simulink model "AXU5EV_PL_Algorithm_Library"  (R2026b)
settings: Solver=VariableStepAuto
libraries: $bdroot x2
settings Model: Creator=lww  LastModifiedBy=lww

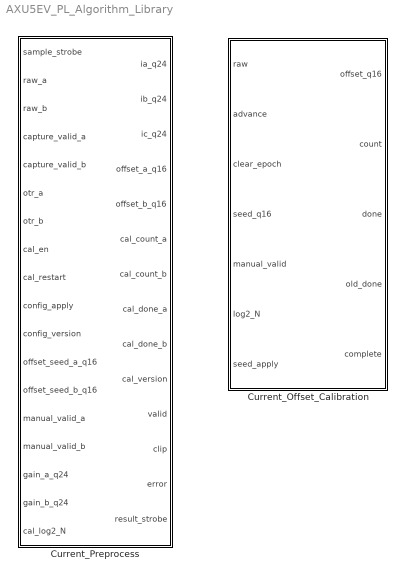
== system AXU5EV_PL_Algorithm_Library ==
  Current_Offset_Calibration : Subsystem  Description=Extracted from the AQM F28335 backup Current_Offset_Calibration (SID350). One independently qualified channel, linked twice for A/B. raw codes -> sum/count -> Q16 offset. Config seeds and log2 window are input ports. Completing sample is rejected using old_done.
  Current_Preprocess : Subsystem  Description=Task1 shared visible current graph. AN9238 Q16 offsets and signed Q24 gains remain atomic input configuration. Independent valid/OTR qualification, wide two-phase reconstruction, convergent rounding and one-clock output registers are preserved.

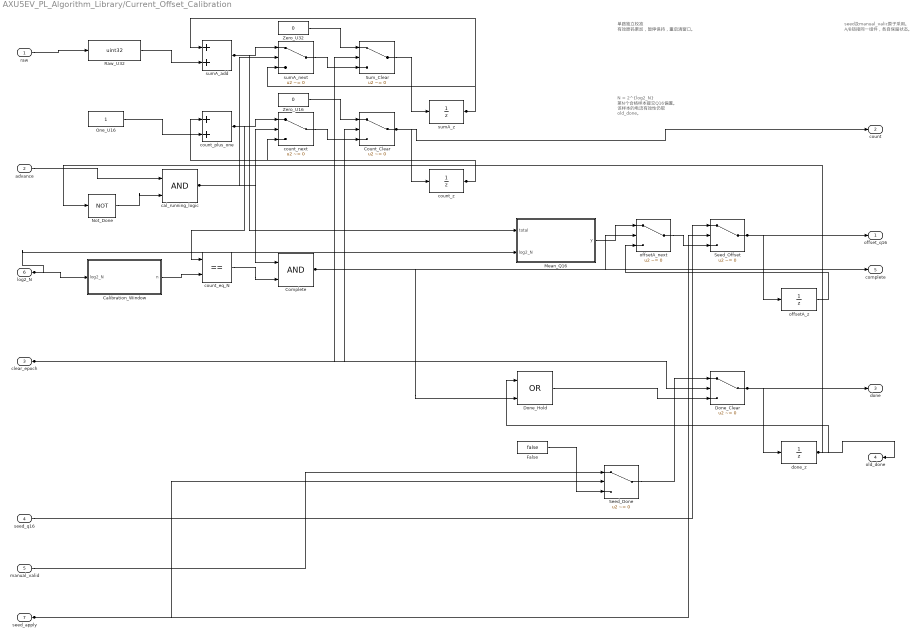
== system AXU5EV_PL_Algorithm_Library/Current_Offset_Calibration ==
  note: seed及manual_valid原子采用。
      | A/B链接同一组件，各自保留状态。
  note: N = 2^{log2_N}
      | 第N个合格样本提交Q16偏置。
      | 该样本的电流有效性仍取 old_done。
  note: 单路独立校准
      | 有效原码累加，暂停保持，重启清窗口。
  raw : Inport  OutDataTypeStr=uint16
  advance : Inport  Port=2  OutDataTypeStr=boolean
  clear_epoch : Inport  Port=3  OutDataTypeStr=boolean
  seed_q16 : Inport  Port=4  OutDataTypeStr=int32
  manual_valid : Inport  Port=5  OutDataTypeStr=boolean
  log2_N : Inport  Port=6  OutDataTypeStr=uint8
  seed_apply : Inport  Port=7  OutDataTypeStr=boolean
  Calibration_Window : MATLAB Function  TreatAsAtomicUnit=on
  Complete : Logic  IconShape=distinctive  AllPortsSameDT=off  OutDataTypeStr=boolean
  Count_Clear : Switch  Criteria=u2 ~= 0  SaturateOnIntegerOverflow=off  InputSameDT=off
  Done_Clear : Switch  Criteria=u2 ~= 0  SaturateOnIntegerOverflow=off  InputSameDT=off
  Done_Hold : Logic  Operator=OR  IconShape=distinctive  AllPortsSameDT=off  OutDataTypeStr=boolean
  False : Constant  Value=false  OutDataTypeStr=boolean
  Mean_Q16 : MATLAB Function  TreatAsAtomicUnit=on
  Not_Done : Logic  Operator=NOT  Inputs=1  IconShape=distinctive  AllPortsSameDT=off  OutDataTypeStr=boolean
  One_U16 : Constant  OutDataTypeStr=uint16
  Raw_U32 : DataTypeConversion  OutDataTypeStr=uint32  SaturateOnIntegerOverflow=off  RndMeth=Floor
  Seed_Done : Switch  Criteria=u2 ~= 0  SaturateOnIntegerOverflow=off  InputSameDT=off
  Seed_Offset : Switch  Criteria=u2 ~= 0  SaturateOnIntegerOverflow=off  InputSameDT=off
  Sum_Clear : Switch  Criteria=u2 ~= 0  SaturateOnIntegerOverflow=off  InputSameDT=off
  Zero_U16 : Constant  Value=0  OutDataTypeStr=uint16
  Zero_U32 : Constant  Value=0  OutDataTypeStr=uint32
  cal_running_logic : Logic  IconShape=distinctive  AllPortsSameDT=off  OutDataTypeStr=boolean
  count_eq_N : RelationalOperator  Operator===  OutDataTypeStr=boolean  RndMeth=Simplest  InputSameDT=off
  count_next : Switch  Criteria=u2 ~= 0  Threshold=0.5  OutDataTypeStr=uint16  SaturateOnIntegerOverflow=off  InputSameDT=off
  count_plus_one : Sum  OutDataTypeStr=uint16
  count_z : UnitDelay  SampleTime=-1
  done_z : UnitDelay  InitialCondition=false  SampleTime=-1
  offsetA_next : Switch  Criteria=u2 ~= 0  Threshold=0.5  OutDataTypeStr=int32  SaturateOnIntegerOverflow=off  InputSameDT=off
  offsetA_z : UnitDelay  SampleTime=-1
  sumA_add : Sum  OutDataTypeStr=uint32
  sumA_next : Switch  Criteria=u2 ~= 0  Threshold=0.5  OutDataTypeStr=uint32  SaturateOnIntegerOverflow=off  InputSameDT=off
  sumA_z : UnitDelay  SampleTime=-1
  offset_q16 : Outport
  count : Outport  Port=2
  done : Outport  Port=3
  old_done : Outport  Port=4
  complete : Outport  Port=5
  wires:
  Done_Clear/1 -> done_z/1, done/1
  Done_Hold/1 -> Done_Clear/3
  Seed_Done/1 -> Done_Clear/1
  False/1 -> Seed_Done/3
  manual_valid/1 -> Seed_Done/1
  Seed_Offset/1 -> offset_q16/1, offsetA_z/1
  seed_apply/1 -> Seed_Offset/2, Seed_Done/2
  seed_q16/1 -> Seed_Offset/1
  Complete/1 -> offsetA_next/2, Done_Hold/2, complete/1
  Mean_Q16/1(y) -> offsetA_next/1
  count_eq_N/1 -> Complete/2
  Calibration_Window/1(n) -> count_eq_N/2
  log2_N/1 -> Calibration_Window/1(log2_N), Mean_Q16/2(log2_N)
  Count_Clear/1 -> count_z/1, count/1
  Sum_Clear/1 -> sumA_z/1
  Zero_U16/1 -> Count_Clear/1
  clear_epoch/1 -> Count_Clear/2, Sum_Clear/2, Done_Clear/2
  Zero_U32/1 -> Sum_Clear/1
  cal_running_logic/1 -> Complete/1, sumA_next/2, count_next/2
  One_U16/1 -> count_plus_one/2
  Raw_U32/1 -> sumA_add/2
  Not_Done/1 -> cal_running_logic/2
  advance/1 -> cal_running_logic/1
  done_z/1 -> old_done/1, Not_Done/1, Done_Hold/1
  offsetA_next/1 -> Seed_Offset/3
  offsetA_z/1 -> offsetA_next/3
  sumA_next/1 -> Sum_Clear/3
  sumA_add/1 -> sumA_next/1, Mean_Q16/1(total)
  raw/1 -> Raw_U32/1
  sumA_z/1 -> sumA_add/1, sumA_next/3
  count_next/1 -> Count_Clear/3
  count_plus_one/1 -> count_next/1, count_eq_N/1
  count_z/1 -> count_plus_one/1, count_next/3

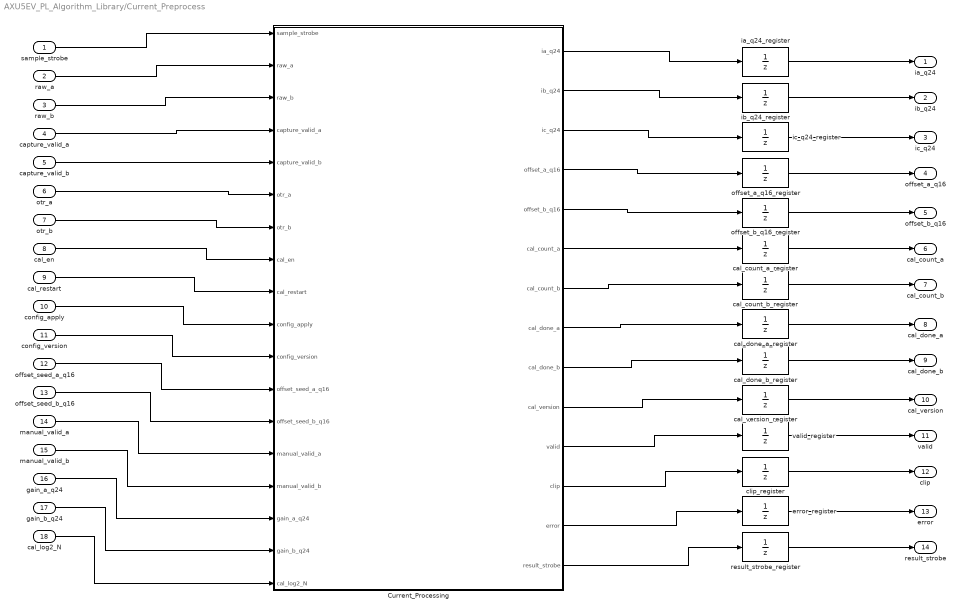
== system AXU5EV_PL_Algorithm_Library/Current_Preprocess ==
  sample_strobe : Inport  OutDataTypeStr=boolean  SampleTime=2e-8
  raw_a : Inport  Port=2  OutDataTypeStr=uint16  SampleTime=2e-8
  raw_b : Inport  Port=3  OutDataTypeStr=uint16  SampleTime=2e-8
  capture_valid_a : Inport  Port=4  OutDataTypeStr=boolean  SampleTime=2e-8
  capture_valid_b : Inport  Port=5  OutDataTypeStr=boolean  SampleTime=2e-8
  otr_a : Inport  Port=6  OutDataTypeStr=boolean  SampleTime=2e-8
  otr_b : Inport  Port=7  OutDataTypeStr=boolean  SampleTime=2e-8
  cal_en : Inport  Port=8  OutDataTypeStr=boolean  SampleTime=2e-8
  cal_restart : Inport  Port=9  OutDataTypeStr=boolean  SampleTime=2e-8
  config_apply : Inport  Port=10  OutDataTypeStr=boolean  SampleTime=2e-8
  config_version : Inport  Port=11  OutDataTypeStr=uint32  SampleTime=2e-8
  offset_seed_a_q16 : Inport  Port=12  OutDataTypeStr=int32  SampleTime=2e-8
  offset_seed_b_q16 : Inport  Port=13  OutDataTypeStr=int32  SampleTime=2e-8
  manual_valid_a : Inport  Port=14  OutDataTypeStr=boolean  SampleTime=2e-8
  manual_valid_b : Inport  Port=15  OutDataTypeStr=boolean  SampleTime=2e-8
  gain_a_q24 : Inport  Port=16  OutDataTypeStr=int32  SampleTime=2e-8
  gain_b_q24 : Inport  Port=17  OutDataTypeStr=int32  SampleTime=2e-8
  cal_log2_N : Inport  Port=18  OutDataTypeStr=uint8  SampleTime=2e-8
  Current_Processing : Subsystem
  cal_count_a_register : UnitDelay  SampleTime=-1
  cal_count_b_register : UnitDelay  SampleTime=-1
  cal_done_a_register : UnitDelay  SampleTime=-1
  cal_done_b_register : UnitDelay  SampleTime=-1
  cal_version_register : UnitDelay  SampleTime=-1
  clip_register : UnitDelay  SampleTime=-1
  error_register : UnitDelay  SampleTime=-1
  ia_q24_register : UnitDelay  SampleTime=-1
  ib_q24_register : UnitDelay  SampleTime=-1
  ic_q24_register : UnitDelay  SampleTime=-1
  offset_a_q16_register : UnitDelay  SampleTime=-1
  offset_b_q16_register : UnitDelay  SampleTime=-1
  result_strobe_register : UnitDelay  SampleTime=-1
  valid_register : UnitDelay  SampleTime=-1
  ia_q24 : Outport  OutDataTypeStr=int32
  ib_q24 : Outport  Port=2  OutDataTypeStr=int32
  ic_q24 : Outport  Port=3  OutDataTypeStr=int32
  offset_a_q16 : Outport  Port=4  OutDataTypeStr=int32
  offset_b_q16 : Outport  Port=5  OutDataTypeStr=int32
  cal_count_a : Outport  Port=6  OutDataTypeStr=uint16
  cal_count_b : Outport  Port=7  OutDataTypeStr=uint16
  cal_done_a : Outport  Port=8  OutDataTypeStr=boolean
  cal_done_b : Outport  Port=9  OutDataTypeStr=boolean
  cal_version : Outport  Port=10  OutDataTypeStr=uint32
  valid : Outport  Port=11  OutDataTypeStr=boolean
  clip : Outport  Port=12  OutDataTypeStr=boolean
  error : Outport  Port=13  OutDataTypeStr=uint16
  result_strobe : Outport  Port=14  OutDataTypeStr=boolean
  wires:
  Current_Processing/14(result_strobe) -> result_strobe_register/1
  Current_Processing/13(error) -> error_register/1
  Current_Processing/12(clip) -> clip_register/1
  Current_Processing/11(valid) -> valid_register/1
  Current_Processing/10(cal_version) -> cal_version_register/1
  Current_Processing/9(cal_done_b) -> cal_done_b_register/1
  Current_Processing/8(cal_done_a) -> cal_done_a_register/1
  Current_Processing/7(cal_count_b) -> cal_count_b_register/1
  Current_Processing/6(cal_count_a) -> cal_count_a_register/1
  Current_Processing/5(offset_b_q16) -> offset_b_q16_register/1
  Current_Processing/4(offset_a_q16) -> offset_a_q16_register/1
  Current_Processing/3(ic_q24) -> ic_q24_register/1
  Current_Processing/2(ib_q24) -> ib_q24_register/1
  Current_Processing/1(ia_q24) -> ia_q24_register/1
  cal_log2_N/1 -> Current_Processing/18(cal_log2_N)
  gain_b_q24/1 -> Current_Processing/17(gain_b_q24)
  gain_a_q24/1 -> Current_Processing/16(gain_a_q24)
  manual_valid_b/1 -> Current_Processing/15(manual_valid_b)
  manual_valid_a/1 -> Current_Processing/14(manual_valid_a)
  offset_seed_b_q16/1 -> Current_Processing/13(offset_seed_b_q16)
  offset_seed_a_q16/1 -> Current_Processing/12(offset_seed_a_q16)
  config_version/1 -> Current_Processing/11(config_version)
  config_apply/1 -> Current_Processing/10(config_apply)
  cal_restart/1 -> Current_Processing/9(cal_restart)
  cal_en/1 -> Current_Processing/8(cal_en)
  otr_b/1 -> Current_Processing/7(otr_b)
  otr_a/1 -> Current_Processing/6(otr_a)
  capture_valid_b/1 -> Current_Processing/5(capture_valid_b)
  capture_valid_a/1 -> Current_Processing/4(capture_valid_a)
  raw_b/1 -> Current_Processing/3(raw_b)
  raw_a/1 -> Current_Processing/2(raw_a)
  sample_strobe/1 -> Current_Processing/1(sample_strobe)
  ia_q24_register/1 -> ia_q24/1
  ib_q24_register/1 -> ib_q24/1
  ic_q24_register/1 -> ic_q24/1
  offset_a_q16_register/1 -> offset_a_q16/1
  offset_b_q16_register/1 -> offset_b_q16/1
  cal_count_a_register/1 -> cal_count_a/1
  cal_count_b_register/1 -> cal_count_b/1
  cal_done_a_register/1 -> cal_done_a/1
  cal_done_b_register/1 -> cal_done_b/1
  cal_version_register/1 -> cal_version/1
  valid_register/1 -> valid/1
  clip_register/1 -> clip/1
  error_register/1 -> error/1
  result_strobe_register/1 -> result_strobe/1

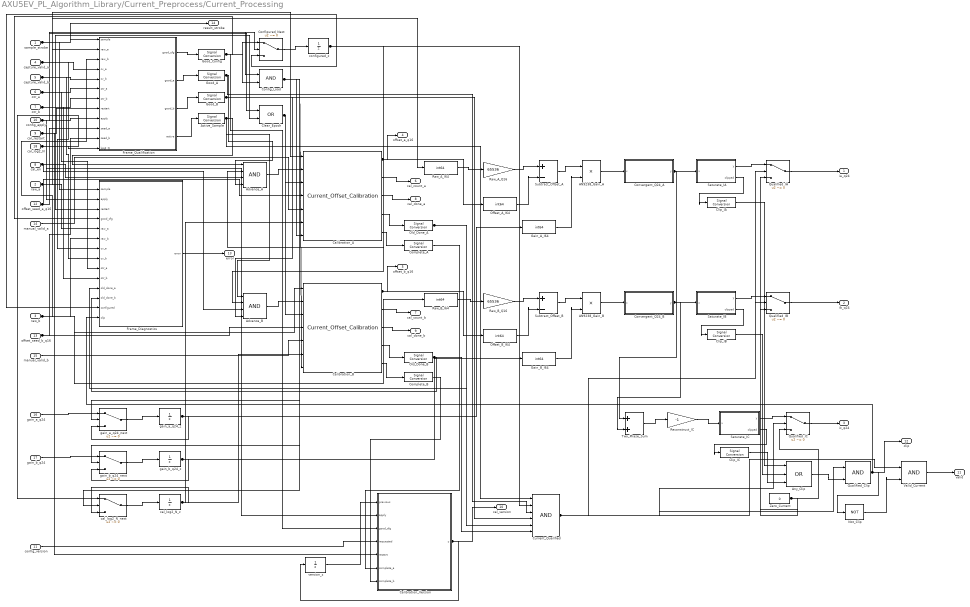
== system AXU5EV_PL_Algorithm_Library/Current_Preprocess/Current_Processing ==
  sample_strobe : Inport
  raw_a : Inport  Port=2
  raw_b : Inport  Port=3
  capture_valid_a : Inport  Port=4
  capture_valid_b : Inport  Port=5
  otr_a : Inport  Port=6
  otr_b : Inport  Port=7
  cal_en : Inport  Port=8
  cal_restart : Inport  Port=9
  config_apply : Inport  Port=10
  config_version : Inport  Port=11
  offset_seed_a_q16 : Inport  Port=12
  offset_seed_b_q16 : Inport  Port=13
  manual_valid_a : Inport  Port=14
  manual_valid_b : Inport  Port=15
  gain_a_q24 : Inport  Port=16
  gain_b_q24 : Inport  Port=17
  cal_log2_N : Inport  Port=18
  AN9238_Gain_A : Product  Inputs=**  OutDataTypeStr=int64
  AN9238_Gain_B : Product  Inputs=**  OutDataTypeStr=int64
  Active_Sample : SignalConversion  OverrideOpt=off
  Advance_A : Logic  Inputs=4  IconShape=distinctive  AllPortsSameDT=off  OutDataTypeStr=boolean
  Advance_B : Logic  Inputs=4  IconShape=distinctive  AllPortsSameDT=off  OutDataTypeStr=boolean
  Any_Clip : Logic  Operator=OR  Inputs=3  IconShape=distinctive  AllPortsSameDT=off  OutDataTypeStr=boolean
  Calibration_A : $bdroot/Current_Offset_Calibration  SystemSampleTime=-1  VariantActivationTime=update diagram  EmptyChoice=off  PassThrough=off  PassThroughVariantControl=(default)  EmptyChoiceVariantControl=(default)  AllowFlexibleInterface=on  Latency=0  AutoFrameSizeCalculation=off
  Calibration_B : $bdroot/Current_Offset_Calibration  SystemSampleTime=-1  VariantActivationTime=update diagram  EmptyChoice=off  PassThrough=off  PassThroughVariantControl=(default)  EmptyChoiceVariantControl=(default)  AllowFlexibleInterface=on  Latency=0  AutoFrameSizeCalculation=off
  Calibration_Version : MATLAB Function  TreatAsAtomicUnit=on
  Clear_Epoch : Logic  Operator=OR  IconShape=distinctive  AllPortsSameDT=off  OutDataTypeStr=boolean
  Clip_IA : SignalConversion  OverrideOpt=off
  Clip_IB : SignalConversion  OverrideOpt=off
  Clip_IC : SignalConversion  OverrideOpt=off
  Complete_A : SignalConversion  OverrideOpt=off
  Complete_B : SignalConversion  OverrideOpt=off
  Config_Load : Logic  IconShape=distinctive  AllPortsSameDT=off  OutDataTypeStr=boolean
  Configured_Next : Switch  Criteria=u2 ~= 0  OutDataTypeStr=boolean  SaturateOnIntegerOverflow=off  InputSameDT=off
  Convergent_Q24_A : MATLAB Function  TreatAsAtomicUnit=on
  Convergent_Q24_B : MATLAB Function  TreatAsAtomicUnit=on
  Current_Qualified : Logic  Inputs=6  IconShape=distinctive  AllPortsSameDT=off  OutDataTypeStr=boolean
  Frame_Diagnostics : MATLAB Function  TreatAsAtomicUnit=on
  Frame_Qualification : MATLAB Function  TreatAsAtomicUnit=on
  Gain_A_I64 : DataTypeConversion  OutDataTypeStr=int64  SaturateOnIntegerOverflow=off  RndMeth=Floor
  Gain_B_I64 : DataTypeConversion  OutDataTypeStr=int64  SaturateOnIntegerOverflow=off  RndMeth=Floor
  Good_A : SignalConversion  OverrideOpt=off
  Good_B : SignalConversion  OverrideOpt=off
  Good_Config : SignalConversion  OverrideOpt=off
  Not_Clip : Logic  Operator=NOT  Inputs=1  IconShape=distinctive  AllPortsSameDT=off  OutDataTypeStr=boolean
  Offset_A_I64 : DataTypeConversion  OutDataTypeStr=int64  SaturateOnIntegerOverflow=off  RndMeth=Floor
  Offset_B_I64 : DataTypeConversion  OutDataTypeStr=int64  SaturateOnIntegerOverflow=off  RndMeth=Floor
  Old_Done_A : SignalConversion  OverrideOpt=off
  Old_Done_B : SignalConversion  OverrideOpt=off
  Qualified_Clip : Logic  IconShape=distinctive  AllPortsSameDT=off  OutDataTypeStr=boolean
  Qualified_IA : Switch  Criteria=u2 ~= 0  SaturateOnIntegerOverflow=off  InputSameDT=off
  Qualified_IB : Switch  Criteria=u2 ~= 0  SaturateOnIntegerOverflow=off  InputSameDT=off
  Qualified_IC : Switch  Criteria=u2 ~= 0  SaturateOnIntegerOverflow=off  InputSameDT=off
  Raw_A_I64 : DataTypeConversion  OutDataTypeStr=int64  SaturateOnIntegerOverflow=off  RndMeth=Floor
  Raw_A_Q16 : Gain  Gain=65536  ParamDataTypeStr=int64  OutDataTypeStr=int64
  Raw_B_I64 : DataTypeConversion  OutDataTypeStr=int64  SaturateOnIntegerOverflow=off  RndMeth=Floor
  Raw_B_Q16 : Gain  Gain=65536  ParamDataTypeStr=int64  OutDataTypeStr=int64
  Reconstruct_IC : Gain  Gain=-1  ParamDataTypeStr=int64  OutDataTypeStr=int64
  Saturate_IA : MATLAB Function  TreatAsAtomicUnit=on
  Saturate_IB : MATLAB Function  TreatAsAtomicUnit=on
  Saturate_IC : MATLAB Function  TreatAsAtomicUnit=on
  Subtract_Offset_A : Sum  Inputs=+-  OutDataTypeStr=int64
  Subtract_Offset_B : Sum  Inputs=+-  OutDataTypeStr=int64
  Two_Phase_Sum : Sum  OutDataTypeStr=int64
  Valid_Current : Logic  IconShape=distinctive  AllPortsSameDT=off  OutDataTypeStr=boolean
  Zero_Current : Constant  Value=0  OutDataTypeStr=int32
  cal_log2_N_next : Switch  Criteria=u2 ~= 0  OutDataTypeStr=uint8  SaturateOnIntegerOverflow=off  InputSameDT=off
  cal_log2_N_z : UnitDelay  InitialCondition=uint8(10)  SampleTime=-1
  configured_z : UnitDelay  InitialCondition=false  SampleTime=-1
  gain_a_q24_next : Switch  Criteria=u2 ~= 0  OutDataTypeStr=int32  SaturateOnIntegerOverflow=off  InputSameDT=off
  gain_a_q24_z : UnitDelay  InitialCondition=int32(0)  SampleTime=-1
  gain_b_q24_next : Switch  Criteria=u2 ~= 0  OutDataTypeStr=int32  SaturateOnIntegerOverflow=off  InputSameDT=off
  gain_b_q24_z : UnitDelay  InitialCondition=int32(0)  SampleTime=-1
  version_z : UnitDelay  InitialCondition=uint32(0)  SampleTime=-1
  ia_q24 : Outport
  ib_q24 : Outport  Port=2
  ic_q24 : Outport  Port=3
  offset_a_q16 : Outport  Port=4
  offset_b_q16 : Outport  Port=5
  cal_count_a : Outport  Port=6
  cal_count_b : Outport  Port=7
  cal_done_a : Outport  Port=8
  cal_done_b : Outport  Port=9
  cal_version : Outport  Port=10
  valid : Outport  Port=11
  clip : Outport  Port=12
  error : Outport  Port=13
  result_strobe : Outport  Port=14
  wires:
  Frame_Diagnostics/1(error) -> error/1
  Calibration_Version/1(y) -> version_z/1, cal_version/1
  Complete_B/1 -> Calibration_Version/7(complete_b)
  Complete_A/1 -> Calibration_Version/6(complete_a)
  config_version/1 -> Calibration_Version/4(requested)
  version_z/1 -> Calibration_Version/1(previous)
  Valid_Current/1 -> valid/1
  Not_Clip/1 -> Valid_Current/2
  Qualified_Clip/1 -> clip/1, Not_Clip/1, Frame_Diagnostics/14(clip)
  Any_Clip/1 -> Qualified_Clip/2
  Clip_IC/1 -> Any_Clip/3
  Clip_IB/1 -> Any_Clip/2
  Clip_IA/1 -> Any_Clip/1
  Saturate_IC/2(clipped) -> Clip_IC/1
  Qualified_IC/1 -> ic_q24/1
  Saturate_IC/1(y) -> Qualified_IC/1
  Reconstruct_IC/1 -> Saturate_IC/1(x)
  Saturate_IB/2(clipped) -> Clip_IB/1
  Qualified_IB/1 -> ib_q24/1
  Saturate_IB/1(y) -> Qualified_IB/1
  Saturate_IA/2(clipped) -> Clip_IA/1
  Qualified_IA/1 -> ia_q24/1
  Zero_Current/1 -> Qualified_IC/3, Qualified_IA/3, Qualified_IB/3
  Current_Qualified/1 -> Qualified_Clip/1, Qualified_IA/2, Qualified_IB/2, Qualified_IC/2, Valid_Current/1
  Saturate_IA/1(y) -> Qualified_IA/1
  Two_Phase_Sum/1 -> Reconstruct_IC/1
  Convergent_Q24_B/1(y) -> Two_Phase_Sum/2, Saturate_IB/1(x)
  Convergent_Q24_A/1(y) -> Two_Phase_Sum/1, Saturate_IA/1(x)
  AN9238_Gain_B/1 -> Convergent_Q24_B/1(x)
  Gain_B_I64/1 -> AN9238_Gain_B/2
  Subtract_Offset_B/1 -> AN9238_Gain_B/1
  Offset_B_I64/1 -> Subtract_Offset_B/2
  Raw_B_Q16/1 -> Subtract_Offset_B/1
  Raw_B_I64/1 -> Raw_B_Q16/1
  AN9238_Gain_A/1 -> Convergent_Q24_A/1(x)
  Gain_A_I64/1 -> AN9238_Gain_A/2
  Subtract_Offset_A/1 -> AN9238_Gain_A/1
  Offset_A_I64/1 -> Subtract_Offset_A/2
  Raw_A_Q16/1 -> Subtract_Offset_A/1
  Raw_A_I64/1 -> Raw_A_Q16/1
  Old_Done_B/1 -> Current_Qualified/6, Frame_Diagnostics/12(old_done_b)
  Old_Done_A/1 -> Current_Qualified/5, Frame_Diagnostics/11(old_done_a)
  Calibration_B/3 -> cal_done_b/1
  Calibration_B/2 -> cal_count_b/1
  Calibration_B/1 -> offset_b_q16/1, Offset_B_I64/1
  Calibration_B/5 -> Complete_B/1
  Calibration_B/4 -> Old_Done_B/1
  manual_valid_b/1 -> Calibration_B/5
  Advance_B/1 -> Calibration_B/2
  Good_B/1 -> Current_Qualified/4, Advance_B/4
  Calibration_A/3 -> cal_done_a/1
  Calibration_A/2 -> cal_count_a/1
  Calibration_A/1 -> Offset_A_I64/1, offset_a_q16/1
  Calibration_A/5 -> Complete_A/1
  Calibration_A/4 -> Old_Done_A/1
  manual_valid_a/1 -> Calibration_A/5
  Clear_Epoch/1 -> Calibration_A/3, Calibration_B/3
  Advance_A/1 -> Calibration_A/2
  Good_A/1 -> Current_Qualified/3, Advance_A/4
  cal_en/1 -> Advance_A/3, Advance_B/3
  Active_Sample/1 -> Advance_A/1, Advance_B/1, Current_Qualified/1
  cal_log2_N_next/1 -> cal_log2_N_z/1
  cal_log2_N_z/1 -> cal_log2_N_next/3, Calibration_A/6, Calibration_B/6
  gain_b_q24_next/1 -> gain_b_q24_z/1
  gain_b_q24_z/1 -> gain_b_q24_next/3, Gain_B_I64/1
  gain_b_q24/1 -> gain_b_q24_next/1
  gain_a_q24_next/1 -> gain_a_q24_z/1
  gain_a_q24_z/1 -> gain_a_q24_next/3, Gain_A_I64/1
  Config_Load/1 -> Calibration_B/7, gain_a_q24_next/2, gain_b_q24_next/2, cal_log2_N_next/2, Calibration_A/7
  gain_a_q24/1 -> gain_a_q24_next/1
  Configured_Next/1 -> configured_z/1
  configured_z/1 -> Configured_Next/3, Current_Qualified/2, Advance_A/2, Advance_B/2, Frame_Diagnostics/13(configured)
  Good_Config/1 -> Frame_Diagnostics/4(good_cfg), Configured_Next/1, Config_Load/2, Calibration_Version/3(good_cfg)
  Frame_Qualification/4(active) -> Active_Sample/1
  Frame_Qualification/3(good_b) -> Good_B/1
  Frame_Qualification/2(good_a) -> Good_A/1
  Frame_Qualification/1(good_cfg) -> Good_Config/1
  cal_log2_N/1 -> Frame_Qualification/12(log2_N), cal_log2_N_next/1
  offset_seed_b_q16/1 -> Calibration_B/4, Frame_Qualification/11(seed_b)
  offset_seed_a_q16/1 -> Calibration_A/4, Frame_Qualification/10(seed_a)
  config_apply/1 -> Calibration_Version/2(apply), Clear_Epoch/1, Config_Load/1, Configured_Next/2, Frame_Qualification/9(apply), Frame_Diagnostics/2(apply)
  cal_restart/1 -> Clear_Epoch/2, Calibration_Version/5(restart), Frame_Qualification/8(restart), Frame_Diagnostics/3(restart)
  otr_b/1 -> Frame_Qualification/7(otr_b), Frame_Diagnostics/10(otr_b)
  otr_a/1 -> Frame_Qualification/6(otr_a), Frame_Diagnostics/9(otr_a)
  capture_valid_b/1 -> Frame_Qualification/5(cv_b), Frame_Diagnostics/8(cv_b)
  capture_valid_a/1 -> Frame_Qualification/4(cv_a), Frame_Diagnostics/7(cv_a)
  raw_b/1 -> Calibration_B/1, Frame_Diagnostics/6(raw_b), Frame_Qualification/3(raw_b), Raw_B_I64/1
  raw_a/1 -> Calibration_A/1, Frame_Diagnostics/5(raw_a), Frame_Qualification/2(raw_a), Raw_A_I64/1
  sample_strobe/1 -> Frame_Diagnostics/1(sample), Frame_Qualification/1(sample), result_strobe/1

== matlab function AXU5EV_PL_Algorithm_Library/Current_Preprocess/Current_Processing/Frame_Diagnostics ==
  data: sample input; error output; apply input; restart input; good_cfg input; raw_a input; raw_b input; cv_a input; cv_b input; otr_a input; otr_b input; old_done_a input; old_done_b input; configured input; clip input
function error=f(sample,apply,restart,good_cfg,raw_a,raw_b,cv_a,cv_b,otr_a,otr_b,old_done_a,old_done_b,configured,clip)
%#codegen
error=uint16(0);
if apply
 if sample,error=uint16(256);end
 if ~good_cfg,error=bitor(error,uint16(64));end
elseif restart
 if sample,error=uint16(256);end
elseif sample
 if ~cv_a || raw_a>uint16(4095),error=bitor(error,uint16(1));end
 if ~cv_b || raw_b>uint16(4095),error=bitor(error,uint16(2));end
 if otr_a,error=bitor(error,uint16(4));end
 if otr_b,error=bitor(error,uint16(8));end
 if ~old_done_a,error=bitor(error,uint16(16));end
 if ~old_done_b,error=bitor(error,uint16(32));end
 if ~configured,error=bitor(error,uint16(64));end
 if clip,error=bitor(error,uint16(128));end
end
end

== matlab function AXU5EV_PL_Algorithm_Library/Current_Offset_Calibration/Mean_Q16 ==
  data: total input; y output; log2_N input
function y=f(total,log2_N)
%#codegen
y=int32(bitshift(uint64(total),int32(16)-int32(log2_N)));
end

== matlab function AXU5EV_PL_Algorithm_Library/Current_Offset_Calibration/Calibration_Window ==
  data: log2_N input; n output
function n=f(log2_N)
%#codegen
n=bitshift(uint16(1),int32(log2_N));
end

== matlab function AXU5EV_PL_Algorithm_Library/Current_Preprocess/Current_Processing/Frame_Qualification ==
  data: sample input; good_cfg output; raw_a input; raw_b input; cv_a input; cv_b input; otr_a input; otr_b input; restart input; apply input; seed_a input; seed_b input; log2_N input; good_a output; good_b output; active output
function [good_cfg,good_a,good_b,active]=f(sample,raw_a,raw_b,cv_a,cv_b,otr_a,otr_b,restart,apply,seed_a,seed_b,log2_N)
%#codegen
limit=int32(268369920);
good_cfg=log2_N<=uint8(10) && seed_a>=int32(0) && seed_a<=limit && seed_b>=int32(0) && seed_b<=limit;
good_a=cv_a && ~otr_a && raw_a<=uint16(4095);
good_b=cv_b && ~otr_b && raw_b<=uint16(4095);
active=sample && ~apply && ~restart;
end

== matlab function AXU5EV_PL_Algorithm_Library/Current_Preprocess/Current_Processing/Convergent_Q24_A ==
  data: x input; y output
function y=f(x)
%#codegen
negative=x<int64(0);a=x;
if negative,a=-x;end
q=bitshift(a,-16);r=bitand(a,int64(65535));
if r>int64(32768) || (r==int64(32768) && bitand(q,int64(1))~=int64(0)),q=q+int64(1);end
if negative,y=-q;else,y=q;end
end

== matlab function AXU5EV_PL_Algorithm_Library/Current_Preprocess/Current_Processing/Convergent_Q24_B ==
  data: x input; y output
function y=f(x)
%#codegen
negative=x<int64(0);a=x;
if negative,a=-x;end
q=bitshift(a,-16);r=bitand(a,int64(65535));
if r>int64(32768) || (r==int64(32768) && bitand(q,int64(1))~=int64(0)),q=q+int64(1);end
if negative,y=-q;else,y=q;end
end

== matlab function AXU5EV_PL_Algorithm_Library/Current_Preprocess/Current_Processing/Saturate_IA ==
  data: x input; y output; clipped output
function [y,clipped]=f(x)
%#codegen
below=bitshift(x,-31)<int64(-1);clipped=x>int64(2147483647)||below;
if x>int64(2147483647),y=int32(2147483647);
elseif below,y=int32(-2147483648);
else,y=int32(x);end
end

== matlab function AXU5EV_PL_Algorithm_Library/Current_Preprocess/Current_Processing/Saturate_IB ==
  data: x input; y output; clipped output
function [y,clipped]=f(x)
%#codegen
below=bitshift(x,-31)<int64(-1);clipped=x>int64(2147483647)||below;
if x>int64(2147483647),y=int32(2147483647);
elseif below,y=int32(-2147483648);
else,y=int32(x);end
end

== matlab function AXU5EV_PL_Algorithm_Library/Current_Preprocess/Current_Processing/Saturate_IC ==
  data: x input; y output; clipped output
function [y,clipped]=f(x)
%#codegen
below=bitshift(x,-31)<int64(-1);clipped=x>int64(2147483647)||below;
if x>int64(2147483647),y=int32(2147483647);
elseif below,y=int32(-2147483648);
else,y=int32(x);end
end

== matlab function AXU5EV_PL_Algorithm_Library/Current_Preprocess/Current_Processing/Calibration_Version ==
  data: previous input; y output; apply input; good_cfg input; requested input; restart input; complete_a input; complete_b input
function y=f(previous,apply,good_cfg,requested,restart,complete_a,complete_b)
%#codegen
y=previous;
if apply
 if good_cfg,y=requested;end
elseif restart
 y=increment(y);
else
 if complete_a,y=increment(y);end
 if complete_b,y=increment(y);end
end
end
function y=increment(x)
if x==uint32(4294967295),y=uint32(0);else,y=x+uint32(1);end
end
